simulink model "ffff"  (R2025a)
settings: Solver=VariableStepAuto  StartTime=0.0  StopTime=16  MaxStep=0.005  RelTol=1e-3
libraries: dspfdesign x1
settings Model: Creator=user  LastModifiedBy=LaL
settings RTWCC: GPUComputeCapability=3.5

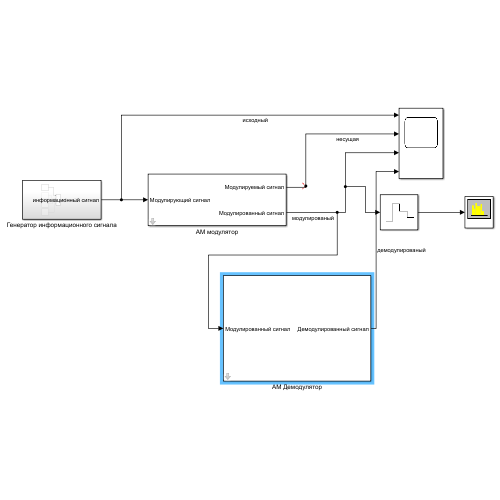
[thumbnail: Simulink's stored preview of the top-level diagram]
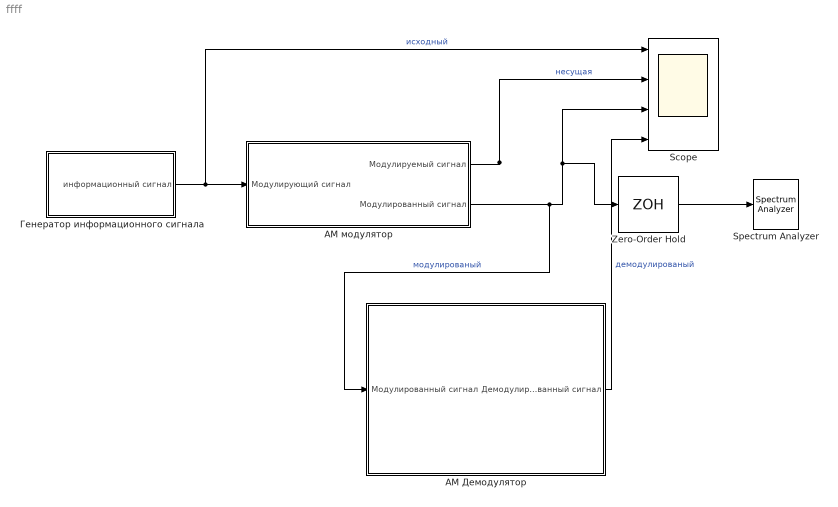
== system ffff ==
  AM модулятор : Subsystem  mask{freq=300, m=0.5}
      mask prompts: freq "Частота несущей"; m "Порядок модуляции"
  Scope : Scope  NumInputPorts=4
      settings: ActiveDisplayYMinimum=-0.31188335263384387  ActiveDisplayYMaximum=0.31188335263384193
  Spectrum Analyzer : SpectrumAnalyzer  WindowPosition=[408.000000,-48.000000,1042.000000,889.000000,]  ScopeFrameLocation=window  SampleRateSource=Property  SampleRate=1000  PlotAsTwoSidedSpectrum=off  StartFrequency=20  StopFrequency=20e3  YLimits=[-177.80889862542756 140.8735902352796]  SelectedToolstripTab=spectrumAnalyzerToolstrip.measurementsTab
  Zero-Order Hold : ZeroOrderHold  SampleTime=1e-3
  АМ Демодулятор : Subsystem  mask{f_c=300}
      mask prompts: f_c "Частота несущей"
  Генератор информационного сигнала : Subsystem
  wires:
  Генератор информационного сигнала/1(информационный сигнал) -> Scope/1, AM модулятор/1(Модулирующий сигнал)  "исходный"
  AM модулятор/1(Модулируемый сигнал) -> Scope/2  "несущая"
  AM модулятор/2(Модулированный сигнал) -> АМ Демодулятор/1(Модулированный сигнал), Scope/3, Zero-Order Hold/1  "модулированый"
  Zero-Order Hold/1 -> Spectrum Analyzer/1
  АМ Демодулятор/1(Демодулированный сигнал) -> Scope/4  "демодулированый"

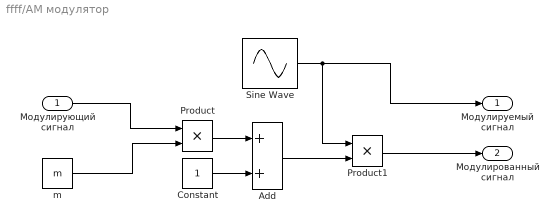
== system ffff/AM модулятор ==
  Модулирующий сигнал : Inport
  Add : Sum
  Constant : Constant
  Product : Product
  Product1 : Product
  Sine Wave : Sin  Frequency=freq*2*pi  SampleTime=0
  m : Constant  Value=m
  Модулируемый сигнал : Outport
  Модулированный сигнал : Outport  Port=2
  wires:
  m/1 -> Product/2
  Модулирующий сигнал/1 -> Product/1
  Product/1 -> Add/1
  Constant/1 -> Add/2
  Sine Wave/1 -> Product1/1, Модулируемый сигнал/1
  Add/1 -> Product1/2
  Product1/1 -> Модулированный сигнал/1

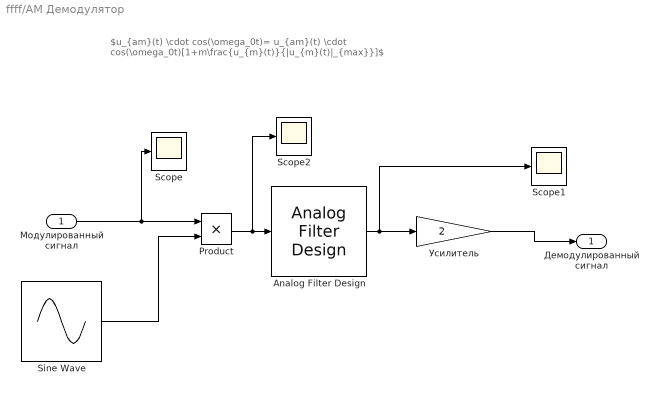
== system ffff/АМ Демодулятор ==
  note: $u_{am}(t) \cdot cos(\omega_0t)= u_{am}(t) \cdot cos(\omega_0t)[1+m\frac{u_{m}(t)}{|u_{m}(t)|_{max}}]$
  Модулированный сигнал : Inport
  Analog Filter Design : dspfdesign/Analog Filter Design  method=Butterworth  filttype=Lowpass  N=16  Wlo=2*pi*f_c  Whi=80  Rp=2  Rs=40
  Product : Product
  Scope : Scope
      settings: ActiveDisplayYMinimum=-1.648911105994975  ActiveDisplayYMaximum=1.6500156220830946
  Scope1 : Scope
      settings: ActiveDisplayYMinimum=-0.045787487676885591  ActiveDisplayYMaximum=0.08243018306325918  DataLoggingVariableName=ScopeData2
  Scope2 : Scope
      settings: ActiveDisplayYMinimum=-1.133357206263194  ActiveDisplayYMaximum=1.032679669776883  DataLoggingVariableName=ScopeData3
  Sine Wave : Sin  Frequency=2*pi*f_c  Phase=pi/2  SampleTime=0
  Усилитель : Gain  Gain=2
  Демодулированный сигнал : Outport
  wires:
  Модулированный сигнал/1 -> Scope/1, Product/1
  Sine Wave/1 -> Product/2
  Product/1 -> Scope2/1, Analog Filter Design/1
  Analog Filter Design/1 -> Scope1/1, Усилитель/1
  Усилитель/1 -> Демодулированный сигнал/1

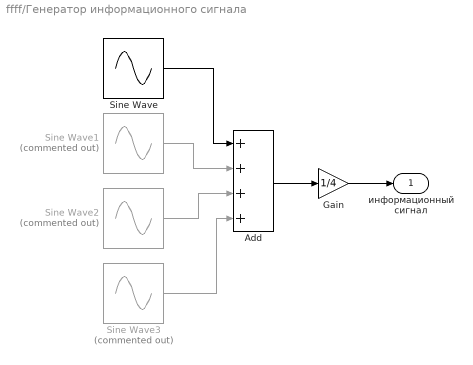
== system ffff/Генератор информационного сигнала ==
  Add : Sum  Inputs=++++
  Gain : Gain  Gain=1/4
  Sine Wave : Sin  Frequency=40*2*pi  SampleTime=0
  Sine Wave1 : Sin  Commented=on  Frequency=60*2*pi  SampleTime=0
  Sine Wave2 : Sin  Commented=on  Frequency=80*2*pi  SampleTime=0
  Sine Wave3 : Sin  Commented=on  Frequency=100*2*pi  SampleTime=0
  информационный сигнал : Outport
  wires:
  Sine Wave1/1 -> Add/2
  Sine Wave2/1 -> Add/3
  Sine Wave3/1 -> Add/4
  Sine Wave/1 -> Add/1
  Add/1 -> Gain/1
  Gain/1 -> информационный сигнал/1
